simulink model "MMC_Per_arm_outer_v5_G2_case1b_delay02_aligned"  (R2024a)
settings: Solver=FixedStepDiscrete  StartTime=0.0  StopTime=2  FixedStep=Ts  RelTol=1e-3
PreLoadFcn:
  | % ---- MMC_Inner4 workspace parameters (control gains live inside the MATLAB Function blocks) ----
  | % ---------------- Converter ----------------
  | VDC     = 800;                  % DC-link voltage (V)  -> Vdc_pos / Vdc_neg = VDC/2
  | N       = 8;                    % submodules per arm
  | C       = 2.2e-3;               % submodule capacitance (F)  -> HB_xx blocks
  | vo      = 100;                  % nominal = initial capacitor voltage (V) = VDC/N  -> HB_xx, Vc_nom
  | W_nom   = 0.5*C*N*vo^2;         % nominal arm energy (J) -> initial condition of the Comm delay blocks
  | Larm    = 5e-3;                 % arm inductance (H)
  | Rarm    = 0.5;                  % arm resistance (ohm)
  | 
  | % ---------------- Grid and PCC filter ----------------
  | f       = 50;                   % grid frequency (Hz)
  | Vg_rms  = 230;                  % grid RMS voltage (V)
  | Vg_pk   = Vg_rms*sqrt(2);       % grid peak voltage (V) -> AC Voltage Source
  | Lg      = 2e-3;                 % line inductance (H)
  | Rg      = 0.1;                  % line resistance (ohm)
  | Cf      = 10e-6;                % AC filter capacitance (F)
  | Rf      = 10;                   % AC filter damping resistance (ohm)
  | 
  | % ---------------- Power set-points ----------------
  | Pstar   = 1500;                 % active-power set-point (W)
  | Qstar   = 0;                    % reactive-power set-point (var)
  | 
  | % ---------------- Timing ----------------
  | fsw     = 1250;                 % carrier frequency per submodule (Hz) -> N*fsw = 10 kHz per arm
  | Ts      = 1e-5;                 % simulation step = submodule-layer step (s)
  | Ts_ctrl = 1e-4;                 % arm-leader control step (s)
  | % ---------------- Test schedule: P* staircase and PCC load (added in _tests) ----------------
  | P_base   = 1500;                % staircase base = first level (W)
  | dP_step  = 250;                 % staircase step (W): 1500 -> 1750 -> 2000 -> 2250 -> 2500
  | t_step   = [0.6 1.0 1.4 1.8];   % step instants (s), 0.4 s hold at each level
  | t_back   = 2.2;                 % return to P_base (s) before the load test
  | P_load1  = 1000;                % PCC load 1 (W at 230 V rms)
  | P_load2  = 1000;                % PCC load 2 (W at 230 V rms)
  | R_load1  = Vg_rms^2/P_load1;    % 52.9 ohm
  | R_load2  = Vg_rms^2/P_load2;    % 52.9 ohm
  | t_load1  = 2.4;                 % Breaker load 1: closes at 2.4 s (stays closed)
  | t_load2  = [2.7 3.0];           % Breaker load 2: closes at 2.7 s, opens at 3.0 s
  | % ---- CASE: twin of case 1 with k_v = 0.2 (balanced start, P* fixed 1500 W, no PCC load, 2 s)
  | % ---- DERIVED: case1b_delay02_aligned: twin + own sample AND neighbour links delayed by 20 samples (0.2 ms), time-aligned
  | % P_SLEW = 5000 W/s, I_max = 17 A, P_max = 2500 W are set INSIDE mmc_outer_ctrl (both arm leaders)
  | t_load1  = 10;  t_load2 = [10 11];   % PCC load test disabled in this case (beyond StopTime)
InitFcn:
  | % ---- MMC_Inner4 workspace parameters (control gains live inside the MATLAB Function blocks) ----
  | % ---------------- Converter ----------------
  | VDC     = 800;                  % DC-link voltage (V)  -> Vdc_pos / Vdc_neg = VDC/2
  | N       = 8;                    % submodules per arm
  | C       = 2.2e-3;               % submodule capacitance (F)  -> HB_xx blocks
  | vo      = 100;                  % nominal = initial capacitor voltage (V) = VDC/N  -> HB_xx, Vc_nom
  | W_nom   = 0.5*C*N*vo^2;         % nominal arm energy (J) -> initial condition of the Comm delay blocks
  | Larm    = 5e-3;                 % arm inductance (H)
  | Rarm    = 0.5;                  % arm resistance (ohm)
  | 
  | % ---------------- Grid and PCC filter ----------------
  | f       = 50;                   % grid frequency (Hz)
  | Vg_rms  = 230;                  % grid RMS voltage (V)
  | Vg_pk   = Vg_rms*sqrt(2);       % grid peak voltage (V) -> AC Voltage Source
  | Lg      = 2e-3;                 % line inductance (H)
  | Rg      = 0.1;                  % line resistance (ohm)
  | Cf      = 10e-6;                % AC filter capacitance (F)
  | Rf      = 10;                   % AC filter damping resistance (ohm)
  | 
  | % ---------------- Power set-points ----------------
  | Pstar   = 1500;                 % active-power set-point (W)
  | Qstar   = 0;                    % reactive-power set-point (var)
  | 
  | % ---------------- Timing ----------------
  | fsw     = 1250;                 % carrier frequency per submodule (Hz) -> N*fsw = 10 kHz per arm
  | Ts      = 1e-5;                 % simulation step = submodule-layer step (s)
  | Ts_ctrl = 1e-4;                 % arm-leader control step (s)
  | % ---------------- Test schedule: P* staircase and PCC load (added in _tests) ----------------
  | P_base   = 1500;                % staircase base = first level (W)
  | dP_step  = 250;                 % staircase step (W): 1500 -> 1750 -> 2000 -> 2250 -> 2500
  | t_step   = [0.6 1.0 1.4 1.8];   % step instants (s), 0.4 s hold at each level
  | t_back   = 2.2;                 % return to P_base (s) before the load test
  | P_load1  = 1000;                % PCC load 1 (W at 230 V rms)
  | P_load2  = 1000;                % PCC load 2 (W at 230 V rms)
  | R_load1  = Vg_rms^2/P_load1;    % 52.9 ohm
  | R_load2  = Vg_rms^2/P_load2;    % 52.9 ohm
  | t_load1  = 2.4;                 % Breaker load 1: closes at 2.4 s (stays closed)
  | t_load2  = [2.7 3.0];           % Breaker load 2: closes at 2.7 s, opens at 3.0 s
  | % ---- CASE: twin of case 1 with k_v = 0.2 (balanced start, P* fixed 1500 W, no PCC load, 2 s)
  | % ---- DERIVED: case1b_delay02_aligned: twin + own sample AND neighbour links delayed by 20 samples (0.2 ms), time-aligned
  | % P_SLEW = 5000 W/s, I_max = 17 A, P_max = 2500 W are set INSIDE mmc_outer_ctrl (both arm leaders)
  | t_load1  = 10;  t_load2 = [10 11];   % PCC load test disabled in this case (beyond StopTime)
libraries: spsHalfBridgeMMCLib x16, spsSeriesRLCBranchLib x6, spsCurrentMeasurementLib x5, spsBreakerLib x2, spsGroundLib x2, spsDCVoltageSourceLib x2, spsACVoltageSourceLib x1, spspowerguiLib x1, spsVoltageMeasurementLib x1
(part 2 of 6)

== matlab function MMC_Per_arm_outer_v5_G2_case1b_delay02_aligned/SM_l3/Neighbors ==
  data: Vc_arm input; Vc_i output; i input; Vc_prev output; Vc_next output
function [Vc_i, Vc_prev, Vc_next] = get_neighbors(Vc_arm, i)
%#codegen
% =========================================================================
% GET_NEIGHBORS  -  Ring-link emulation for submodule number i
% -------------------------------------------------------------------------
% Block     : "Neighbors" inside every SM_ux / SM_lx subsystem
% Rate      : Ts = 10 us
% Instances : 16 (one per submodule)
% Purpose   : in simulation the whole capacitor-voltage vector of the arm is
%             available, but a real submodule only knows its OWN voltage and
%             the voltages of its two ring neighbours. This block hides
%             everything else, so the local controller stays truly local.
% Inputs    : Vc_arm  N x 1 vector of capacitor voltages of the arm (V)
%             i       own submodule index, 1..N
% Outputs   : Vc_i    own capacitor voltage (V)
%             Vc_prev voltage of the previous ring neighbour (V)
%             Vc_next voltage of the next ring neighbour (V)
% =========================================================================

%% ---------------- PARAMETERS ----------------
N = 8;                                   % submodules per arm (= length of Vc_arm, the Mux of the 8 HB voltages)
ND = 20;                              % ALIGNED-DELAY case: own AND neighbour values delayed by ND samples (Ts = 10 us -> 0.2 ms)
persistent buf_i buf_p buf_n idx         % circular buffers of the own sample and the two neighbour links, and the index

%% ---------------- 1. own index, made safe ----------------
k = min(max(round(i), 1), N);            % round to an integer and clamp to [1, N] (protects against a bad sm_id)

%% ---------------- 2. own voltage ----------------
Vc_i = Vc_arm(k);                        % own capacitor voltage

%% ---------------- 3. ring neighbours (circular: SM1 and SMN are neighbours) ----------------
if k == 1                                % first submodule of the ring
    Vc_prev = Vc_arm(N);                 % previous neighbour wraps around to the last submodule
    Vc_next = Vc_arm(2);                 % next neighbour is SM2
elseif k == N                            % last submodule of the ring
    Vc_prev = Vc_arm(N - 1);             % previous neighbour is SM(N-1)
    Vc_next = Vc_arm(1);                 % next neighbour wraps around to SM1
else                                     % any submodule in the middle
    Vc_prev = Vc_arm(k - 1);             % previous neighbour
    Vc_next = Vc_arm(k + 1);             % next neighbour
end

%% ---------------- 4. time-aligned delay: own sample and neighbour links delayed by the same ND (ALIGNED-DELAY case) ----------------
if isempty(buf_i)                        % first call
    buf_i = Vc_i    * ones(ND, 1);       % buffers start filled with the first values: no false error during the first ND samples
    buf_p = Vc_prev * ones(ND, 1);
    buf_n = Vc_next * ones(ND, 1);
    idx   = 1;
end
d_i    = buf_i(idx);                     % own voltage ND samples ago (same instant as the neighbour values)
d_prev = buf_p(idx);                     % value sent by the previous neighbour ND samples ago
d_next = buf_n(idx);                     % value sent by the next neighbour ND samples ago
buf_i(idx) = Vc_i;                       % store the fresh values in the slot just read
buf_p(idx) = Vc_prev;
buf_n(idx) = Vc_next;
idx = idx + 1;                           % advance the circular index
if idx > ND
    idx = 1;
end
Vc_i    = d_i;                           % the local controller compares three values of the SAME instant t - tau
Vc_prev = d_prev;
Vc_next = d_next;
end

== matlab function MMC_Per_arm_outer_v5_G2_case1b_delay02_aligned/SM_l3/Local Ctrl ==
  data: sm_id input; S_top output; m_arm input; i_arm input; Vc_i input; Vc_prev input; Vc_next input; t input; S_bot output
function [S_top, S_bot] = hb_sm_local_ctrl(sm_id, m_arm, i_arm, Vc_i, Vc_prev, Vc_next, t)
%#codegen
% =========================================================================
% HB_SM_LOCAL_CTRL  -  Submodule local controller: neighbour balancing + PSC-PWM
% -------------------------------------------------------------------------
% Block     : "Local Ctrl" inside every SM_ux / SM_lx subsystem
% Rate      : Ts = 10 us
% Instances : 16 (one per half-bridge submodule)
% Purpose   : decide the two gate signals of ONE half-bridge submodule using
%             only local information: own capacitor voltage, the two ring
%             neighbours, the arm modulation index sent by the arm leader,
%             the arm-current direction and the time base.
%             No sorting and no access to the full capacitor-voltage vector.
% Inputs    : sm_id    own index 1..N (sets the carrier phase shift)
%             m_arm    arm modulation index from the arm leader, in [0, 1]
%             i_arm    arm current (A), only its direction is used
%             Vc_i     own capacitor voltage (V)
%             Vc_prev  previous ring neighbour voltage (V)
%             Vc_next  next ring neighbour voltage (V)
%             t        simulation time (s), carrier time base
% Outputs   : S_top    upper switch gate (1 = on)  -> capacitor INSERTED (+Vc)
%             S_bot    lower switch gate (1 = on)  -> capacitor BYPASSED (0 V)
% =========================================================================

%% ---------------- PARAMETERS ----------------
N      = 8;                              % submodules per arm -> carrier phase shift of SM k = (k-1)/N of a period
fsw    = 1250;                           % carrier frequency per submodule (Hz) -> N*fsw = 10 kHz apparent arm ripple
k_v    = 0.2;                            % balancing gain (1/V): modulation-index change per volt of error
dead   = 0.1;                            % dead-band (V): errors smaller than this are ignored (no chattering)
Iscale = 1.0;                            % current scale (A) of the smooth sign function tanh(i_arm/Iscale)

%% ---------------- 1. neighbour-average balancing correction ----------------
err  = 0.5*(Vc_prev + Vc_next) - Vc_i;   % error = neighbour average - own voltage (> 0: I am too low, I need charging)
if abs(err) < dead                       % error inside the dead-band?
    err = 0;                             % ignore it
end
dirn = tanh(i_arm / Iscale);             % smooth current direction in (-1, +1); > 0 means inserting CHARGES the capacitor
dm   = k_v * err * dirn;                 % correction: insert more if charging is needed AND the current charges, less otherwise
m_i  = min(max(m_arm + dm, 0), 1);       % own modulation index = arm index + correction, clamped to [0, 1]

%% ---------------- 2. phase-shifted triangular carrier (0 -> 1 -> 0) ----------------
tau = mod(t*fsw + (sm_id - 1)/N, 1);     % position inside the carrier period, in [0, 1), shifted by (sm_id-1)/N
car = 1 - abs(2*tau - 1);                % triangle: rises 0 -> 1 on the first half, falls 1 -> 0 on the second half

%% ---------------- 3. half-bridge gating ----------------
if m_i >= car                            % modulation index above the carrier?
    S_top = 1;                           % upper switch on  -> capacitor inserted (+Vc on the arm)
    S_bot = 0;                           % lower switch off
else                                     % modulation index below the carrier
    S_top = 0;                           % upper switch off
    S_bot = 1;                           % lower switch on  -> capacitor bypassed (0 V)
end
end

== matlab function MMC_Per_arm_outer_v5_G2_case1b_delay02_aligned/SM_u4/Neighbors ==
  data: Vc_arm input; Vc_i output; i input; Vc_prev output; Vc_next output
function [Vc_i, Vc_prev, Vc_next] = get_neighbors(Vc_arm, i)
%#codegen
% =========================================================================
% GET_NEIGHBORS  -  Ring-link emulation for submodule number i
% -------------------------------------------------------------------------
% Block     : "Neighbors" inside every SM_ux / SM_lx subsystem
% Rate      : Ts = 10 us
% Instances : 16 (one per submodule)
% Purpose   : in simulation the whole capacitor-voltage vector of the arm is
%             available, but a real submodule only knows its OWN voltage and
%             the voltages of its two ring neighbours. This block hides
%             everything else, so the local controller stays truly local.
% Inputs    : Vc_arm  N x 1 vector of capacitor voltages of the arm (V)
%             i       own submodule index, 1..N
% Outputs   : Vc_i    own capacitor voltage (V)
%             Vc_prev voltage of the previous ring neighbour (V)
%             Vc_next voltage of the next ring neighbour (V)
% =========================================================================

%% ---------------- PARAMETERS ----------------
N = 8;                                   % submodules per arm (= length of Vc_arm, the Mux of the 8 HB voltages)
ND = 20;                              % ALIGNED-DELAY case: own AND neighbour values delayed by ND samples (Ts = 10 us -> 0.2 ms)
persistent buf_i buf_p buf_n idx         % circular buffers of the own sample and the two neighbour links, and the index

%% ---------------- 1. own index, made safe ----------------
k = min(max(round(i), 1), N);            % round to an integer and clamp to [1, N] (protects against a bad sm_id)

%% ---------------- 2. own voltage ----------------
Vc_i = Vc_arm(k);                        % own capacitor voltage

%% ---------------- 3. ring neighbours (circular: SM1 and SMN are neighbours) ----------------
if k == 1                                % first submodule of the ring
    Vc_prev = Vc_arm(N);                 % previous neighbour wraps around to the last submodule
    Vc_next = Vc_arm(2);                 % next neighbour is SM2
elseif k == N                            % last submodule of the ring
    Vc_prev = Vc_arm(N - 1);             % previous neighbour is SM(N-1)
    Vc_next = Vc_arm(1);                 % next neighbour wraps around to SM1
else                                     % any submodule in the middle
    Vc_prev = Vc_arm(k - 1);             % previous neighbour
    Vc_next = Vc_arm(k + 1);             % next neighbour
end

%% ---------------- 4. time-aligned delay: own sample and neighbour links delayed by the same ND (ALIGNED-DELAY case) ----------------
if isempty(buf_i)                        % first call
    buf_i = Vc_i    * ones(ND, 1);       % buffers start filled with the first values: no false error during the first ND samples
    buf_p = Vc_prev * ones(ND, 1);
    buf_n = Vc_next * ones(ND, 1);
    idx   = 1;
end
d_i    = buf_i(idx);                     % own voltage ND samples ago (same instant as the neighbour values)
d_prev = buf_p(idx);                     % value sent by the previous neighbour ND samples ago
d_next = buf_n(idx);                     % value sent by the next neighbour ND samples ago
buf_i(idx) = Vc_i;                       % store the fresh values in the slot just read
buf_p(idx) = Vc_prev;
buf_n(idx) = Vc_next;
idx = idx + 1;                           % advance the circular index
if idx > ND
    idx = 1;
end
Vc_i    = d_i;                           % the local controller compares three values of the SAME instant t - tau
Vc_prev = d_prev;
Vc_next = d_next;
end

== matlab function MMC_Per_arm_outer_v5_G2_case1b_delay02_aligned/SM_u1/Local Ctrl ==
  data: sm_id input; S_top output; m_arm input; i_arm input; Vc_i input; Vc_prev input; Vc_next input; t input; S_bot output
function [S_top, S_bot] = hb_sm_local_ctrl(sm_id, m_arm, i_arm, Vc_i, Vc_prev, Vc_next, t)
%#codegen
% =========================================================================
% HB_SM_LOCAL_CTRL  -  Submodule local controller: neighbour balancing + PSC-PWM
% -------------------------------------------------------------------------
% Block     : "Local Ctrl" inside every SM_ux / SM_lx subsystem
% Rate      : Ts = 10 us
% Instances : 16 (one per half-bridge submodule)
% Purpose   : decide the two gate signals of ONE half-bridge submodule using
%             only local information: own capacitor voltage, the two ring
%             neighbours, the arm modulation index sent by the arm leader,
%             the arm-current direction and the time base.
%             No sorting and no access to the full capacitor-voltage vector.
% Inputs    : sm_id    own index 1..N (sets the carrier phase shift)
%             m_arm    arm modulation index from the arm leader, in [0, 1]
%             i_arm    arm current (A), only its direction is used
%             Vc_i     own capacitor voltage (V)
%             Vc_prev  previous ring neighbour voltage (V)
%             Vc_next  next ring neighbour voltage (V)
%             t        simulation time (s), carrier time base
% Outputs   : S_top    upper switch gate (1 = on)  -> capacitor INSERTED (+Vc)
%             S_bot    lower switch gate (1 = on)  -> capacitor BYPASSED (0 V)
% =========================================================================

%% ---------------- PARAMETERS ----------------
N      = 8;                              % submodules per arm -> carrier phase shift of SM k = (k-1)/N of a period
fsw    = 1250;                           % carrier frequency per submodule (Hz) -> N*fsw = 10 kHz apparent arm ripple
k_v    = 0.2;                            % balancing gain (1/V): modulation-index change per volt of error
dead   = 0.1;                            % dead-band (V): errors smaller than this are ignored (no chattering)
Iscale = 1.0;                            % current scale (A) of the smooth sign function tanh(i_arm/Iscale)

%% ---------------- 1. neighbour-average balancing correction ----------------
err  = 0.5*(Vc_prev + Vc_next) - Vc_i;   % error = neighbour average - own voltage (> 0: I am too low, I need charging)
if abs(err) < dead                       % error inside the dead-band?
    err = 0;                             % ignore it
end
dirn = tanh(i_arm / Iscale);             % smooth current direction in (-1, +1); > 0 means inserting CHARGES the capacitor
dm   = k_v * err * dirn;                 % correction: insert more if charging is needed AND the current charges, less otherwise
m_i  = min(max(m_arm + dm, 0), 1);       % own modulation index = arm index + correction, clamped to [0, 1]

%% ---------------- 2. phase-shifted triangular carrier (0 -> 1 -> 0) ----------------
tau = mod(t*fsw + (sm_id - 1)/N, 1);     % position inside the carrier period, in [0, 1), shifted by (sm_id-1)/N
car = 1 - abs(2*tau - 1);                % triangle: rises 0 -> 1 on the first half, falls 1 -> 0 on the second half

%% ---------------- 3. half-bridge gating ----------------
if m_i >= car                            % modulation index above the carrier?
    S_top = 1;                           % upper switch on  -> capacitor inserted (+Vc on the arm)
    S_bot = 0;                           % lower switch off
else                                     % modulation index below the carrier
    S_top = 0;                           % upper switch off
    S_bot = 1;                           % lower switch on  -> capacitor bypassed (0 V)
end
end

== matlab function MMC_Per_arm_outer_v5_G2_case1b_delay02_aligned/SM_u4/Local Ctrl ==
  data: sm_id input; S_top output; m_arm input; i_arm input; Vc_i input; Vc_prev input; Vc_next input; t input; S_bot output
function [S_top, S_bot] = hb_sm_local_ctrl(sm_id, m_arm, i_arm, Vc_i, Vc_prev, Vc_next, t)
%#codegen
% =========================================================================
% HB_SM_LOCAL_CTRL  -  Submodule local controller: neighbour balancing + PSC-PWM
% -------------------------------------------------------------------------
% Block     : "Local Ctrl" inside every SM_ux / SM_lx subsystem
% Rate      : Ts = 10 us
% Instances : 16 (one per half-bridge submodule)
% Purpose   : decide the two gate signals of ONE half-bridge submodule using
%             only local information: own capacitor voltage, the two ring
%             neighbours, the arm modulation index sent by the arm leader,
%             the arm-current direction and the time base.
%             No sorting and no access to the full capacitor-voltage vector.
% Inputs    : sm_id    own index 1..N (sets the carrier phase shift)
%             m_arm    arm modulation index from the arm leader, in [0, 1]
%             i_arm    arm current (A), only its direction is used
%             Vc_i     own capacitor voltage (V)
%             Vc_prev  previous ring neighbour voltage (V)
%             Vc_next  next ring neighbour voltage (V)
%             t        simulation time (s), carrier time base
% Outputs   : S_top    upper switch gate (1 = on)  -> capacitor INSERTED (+Vc)
%             S_bot    lower switch gate (1 = on)  -> capacitor BYPASSED (0 V)
% =========================================================================

%% ---------------- PARAMETERS ----------------
N      = 8;                              % submodules per arm -> carrier phase shift of SM k = (k-1)/N of a period
fsw    = 1250;                           % carrier frequency per submodule (Hz) -> N*fsw = 10 kHz apparent arm ripple
k_v    = 0.2;                            % balancing gain (1/V): modulation-index change per volt of error
dead   = 0.1;                            % dead-band (V): errors smaller than this are ignored (no chattering)
Iscale = 1.0;                            % current scale (A) of the smooth sign function tanh(i_arm/Iscale)

%% ---------------- 1. neighbour-average balancing correction ----------------
err  = 0.5*(Vc_prev + Vc_next) - Vc_i;   % error = neighbour average - own voltage (> 0: I am too low, I need charging)
if abs(err) < dead                       % error inside the dead-band?
    err = 0;                             % ignore it
end
dirn = tanh(i_arm / Iscale);             % smooth current direction in (-1, +1); > 0 means inserting CHARGES the capacitor
dm   = k_v * err * dirn;                 % correction: insert more if charging is needed AND the current charges, less otherwise
m_i  = min(max(m_arm + dm, 0), 1);       % own modulation index = arm index + correction, clamped to [0, 1]

%% ---------------- 2. phase-shifted triangular carrier (0 -> 1 -> 0) ----------------
tau = mod(t*fsw + (sm_id - 1)/N, 1);     % position inside the carrier period, in [0, 1), shifted by (sm_id-1)/N
car = 1 - abs(2*tau - 1);                % triangle: rises 0 -> 1 on the first half, falls 1 -> 0 on the second half

%% ---------------- 3. half-bridge gating ----------------
if m_i >= car                            % modulation index above the carrier?
    S_top = 1;                           % upper switch on  -> capacitor inserted (+Vc on the arm)
    S_bot = 0;                           % lower switch off
else                                     % modulation index below the carrier
    S_top = 0;                           % upper switch off
    S_bot = 1;                           % lower switch on  -> capacitor bypassed (0 V)
end
end

== matlab function MMC_Per_arm_outer_v5_G2_case1b_delay02_aligned/SM_l4/Neighbors ==
  data: Vc_arm input; Vc_i output; i input; Vc_prev output; Vc_next output
function [Vc_i, Vc_prev, Vc_next] = get_neighbors(Vc_arm, i)
%#codegen
% =========================================================================
% GET_NEIGHBORS  -  Ring-link emulation for submodule number i
% -------------------------------------------------------------------------
% Block     : "Neighbors" inside every SM_ux / SM_lx subsystem
% Rate      : Ts = 10 us
% Instances : 16 (one per submodule)
% Purpose   : in simulation the whole capacitor-voltage vector of the arm is
%             available, but a real submodule only knows its OWN voltage and
%             the voltages of its two ring neighbours. This block hides
%             everything else, so the local controller stays truly local.
% Inputs    : Vc_arm  N x 1 vector of capacitor voltages of the arm (V)
%             i       own submodule index, 1..N
% Outputs   : Vc_i    own capacitor voltage (V)
%             Vc_prev voltage of the previous ring neighbour (V)
%             Vc_next voltage of the next ring neighbour (V)
% =========================================================================

%% ---------------- PARAMETERS ----------------
N = 8;                                   % submodules per arm (= length of Vc_arm, the Mux of the 8 HB voltages)
ND = 20;                              % ALIGNED-DELAY case: own AND neighbour values delayed by ND samples (Ts = 10 us -> 0.2 ms)
persistent buf_i buf_p buf_n idx         % circular buffers of the own sample and the two neighbour links, and the index

%% ---------------- 1. own index, made safe ----------------
k = min(max(round(i), 1), N);            % round to an integer and clamp to [1, N] (protects against a bad sm_id)

%% ---------------- 2. own voltage ----------------
Vc_i = Vc_arm(k);                        % own capacitor voltage

%% ---------------- 3. ring neighbours (circular: SM1 and SMN are neighbours) ----------------
if k == 1                                % first submodule of the ring
    Vc_prev = Vc_arm(N);                 % previous neighbour wraps around to the last submodule
    Vc_next = Vc_arm(2);                 % next neighbour is SM2
elseif k == N                            % last submodule of the ring
    Vc_prev = Vc_arm(N - 1);             % previous neighbour is SM(N-1)
    Vc_next = Vc_arm(1);                 % next neighbour wraps around to SM1
else                                     % any submodule in the middle
    Vc_prev = Vc_arm(k - 1);             % previous neighbour
    Vc_next = Vc_arm(k + 1);             % next neighbour
end

%% ---------------- 4. time-aligned delay: own sample and neighbour links delayed by the same ND (ALIGNED-DELAY case) ----------------
if isempty(buf_i)                        % first call
    buf_i = Vc_i    * ones(ND, 1);       % buffers start filled with the first values: no false error during the first ND samples
    buf_p = Vc_prev * ones(ND, 1);
    buf_n = Vc_next * ones(ND, 1);
    idx   = 1;
end
d_i    = buf_i(idx);                     % own voltage ND samples ago (same instant as the neighbour values)
d_prev = buf_p(idx);                     % value sent by the previous neighbour ND samples ago
d_next = buf_n(idx);                     % value sent by the next neighbour ND samples ago
buf_i(idx) = Vc_i;                       % store the fresh values in the slot just read
buf_p(idx) = Vc_prev;
buf_n(idx) = Vc_next;
idx = idx + 1;                           % advance the circular index
if idx > ND
    idx = 1;
end
Vc_i    = d_i;                           % the local controller compares three values of the SAME instant t - tau
Vc_prev = d_prev;
Vc_next = d_next;
end

== matlab function MMC_Per_arm_outer_v5_G2_case1b_delay02_aligned/SM_l4/Local Ctrl ==
  data: sm_id input; S_top output; m_arm input; i_arm input; Vc_i input; Vc_prev input; Vc_next input; t input; S_bot output
function [S_top, S_bot] = hb_sm_local_ctrl(sm_id, m_arm, i_arm, Vc_i, Vc_prev, Vc_next, t)
%#codegen
% =========================================================================
% HB_SM_LOCAL_CTRL  -  Submodule local controller: neighbour balancing + PSC-PWM
% -------------------------------------------------------------------------
% Block     : "Local Ctrl" inside every SM_ux / SM_lx subsystem
% Rate      : Ts = 10 us
% Instances : 16 (one per half-bridge submodule)
% Purpose   : decide the two gate signals of ONE half-bridge submodule using
%             only local information: own capacitor voltage, the two ring
%             neighbours, the arm modulation index sent by the arm leader,
%             the arm-current direction and the time base.
%             No sorting and no access to the full capacitor-voltage vector.
% Inputs    : sm_id    own index 1..N (sets the carrier phase shift)
%             m_arm    arm modulation index from the arm leader, in [0, 1]
%             i_arm    arm current (A), only its direction is used
%             Vc_i     own capacitor voltage (V)
%             Vc_prev  previous ring neighbour voltage (V)
%             Vc_next  next ring neighbour voltage (V)
%             t        simulation time (s), carrier time base
% Outputs   : S_top    upper switch gate (1 = on)  -> capacitor INSERTED (+Vc)
%             S_bot    lower switch gate (1 = on)  -> capacitor BYPASSED (0 V)
% =========================================================================

%% ---------------- PARAMETERS ----------------
N      = 8;                              % submodules per arm -> carrier phase shift of SM k = (k-1)/N of a period
fsw    = 1250;                           % carrier frequency per submodule (Hz) -> N*fsw = 10 kHz apparent arm ripple
k_v    = 0.2;                            % balancing gain (1/V): modulation-index change per volt of error
dead   = 0.1;                            % dead-band (V): errors smaller than this are ignored (no chattering)
Iscale = 1.0;                            % current scale (A) of the smooth sign function tanh(i_arm/Iscale)

%% ---------------- 1. neighbour-average balancing correction ----------------
err  = 0.5*(Vc_prev + Vc_next) - Vc_i;   % error = neighbour average - own voltage (> 0: I am too low, I need charging)
if abs(err) < dead                       % error inside the dead-band?
    err = 0;                             % ignore it
end
dirn = tanh(i_arm / Iscale);             % smooth current direction in (-1, +1); > 0 means inserting CHARGES the capacitor
dm   = k_v * err * dirn;                 % correction: insert more if charging is needed AND the current charges, less otherwise
m_i  = min(max(m_arm + dm, 0), 1);       % own modulation index = arm index + correction, clamped to [0, 1]

%% ---------------- 2. phase-shifted triangular carrier (0 -> 1 -> 0) ----------------
tau = mod(t*fsw + (sm_id - 1)/N, 1);     % position inside the carrier period, in [0, 1), shifted by (sm_id-1)/N
car = 1 - abs(2*tau - 1);                % triangle: rises 0 -> 1 on the first half, falls 1 -> 0 on the second half

%% ---------------- 3. half-bridge gating ----------------
if m_i >= car                            % modulation index above the carrier?
    S_top = 1;                           % upper switch on  -> capacitor inserted (+Vc on the arm)
    S_bot = 0;                           % lower switch off
else                                     % modulation index below the carrier
    S_top = 0;                           % upper switch off
    S_bot = 1;                           % lower switch on  -> capacitor bypassed (0 V)
end
end

== matlab function MMC_Per_arm_outer_v5_G2_case1b_delay02_aligned/SM_u5/Neighbors ==
  data: Vc_arm input; Vc_i output; i input; Vc_prev output; Vc_next output
function [Vc_i, Vc_prev, Vc_next] = get_neighbors(Vc_arm, i)
%#codegen
% =========================================================================
% GET_NEIGHBORS  -  Ring-link emulation for submodule number i
% -------------------------------------------------------------------------
% Block     : "Neighbors" inside every SM_ux / SM_lx subsystem
% Rate      : Ts = 10 us
% Instances : 16 (one per submodule)
% Purpose   : in simulation the whole capacitor-voltage vector of the arm is
%             available, but a real submodule only knows its OWN voltage and
%             the voltages of its two ring neighbours. This block hides
%             everything else, so the local controller stays truly local.
% Inputs    : Vc_arm  N x 1 vector of capacitor voltages of the arm (V)
%             i       own submodule index, 1..N
% Outputs   : Vc_i    own capacitor voltage (V)
%             Vc_prev voltage of the previous ring neighbour (V)
%             Vc_next voltage of the next ring neighbour (V)
% =========================================================================

%% ---------------- PARAMETERS ----------------
N = 8;                                   % submodules per arm (= length of Vc_arm, the Mux of the 8 HB voltages)
ND = 20;                              % ALIGNED-DELAY case: own AND neighbour values delayed by ND samples (Ts = 10 us -> 0.2 ms)
persistent buf_i buf_p buf_n idx         % circular buffers of the own sample and the two neighbour links, and the index

%% ---------------- 1. own index, made safe ----------------
k = min(max(round(i), 1), N);            % round to an integer and clamp to [1, N] (protects against a bad sm_id)

%% ---------------- 2. own voltage ----------------
Vc_i = Vc_arm(k);                        % own capacitor voltage

%% ---------------- 3. ring neighbours (circular: SM1 and SMN are neighbours) ----------------
if k == 1                                % first submodule of the ring
    Vc_prev = Vc_arm(N);                 % previous neighbour wraps around to the last submodule
    Vc_next = Vc_arm(2);                 % next neighbour is SM2
elseif k == N                            % last submodule of the ring
    Vc_prev = Vc_arm(N - 1);             % previous neighbour is SM(N-1)
    Vc_next = Vc_arm(1);                 % next neighbour wraps around to SM1
else                                     % any submodule in the middle
    Vc_prev = Vc_arm(k - 1);             % previous neighbour
    Vc_next = Vc_arm(k + 1);             % next neighbour
end

%% ---------------- 4. time-aligned delay: own sample and neighbour links delayed by the same ND (ALIGNED-DELAY case) ----------------
if isempty(buf_i)                        % first call
    buf_i = Vc_i    * ones(ND, 1);       % buffers start filled with the first values: no false error during the first ND samples
    buf_p = Vc_prev * ones(ND, 1);
    buf_n = Vc_next * ones(ND, 1);
    idx   = 1;
end
d_i    = buf_i(idx);                     % own voltage ND samples ago (same instant as the neighbour values)
d_prev = buf_p(idx);                     % value sent by the previous neighbour ND samples ago
d_next = buf_n(idx);                     % value sent by the next neighbour ND samples ago
buf_i(idx) = Vc_i;                       % store the fresh values in the slot just read
buf_p(idx) = Vc_prev;
buf_n(idx) = Vc_next;
idx = idx + 1;                           % advance the circular index
if idx > ND
    idx = 1;
end
Vc_i    = d_i;                           % the local controller compares three values of the SAME instant t - tau
Vc_prev = d_prev;
Vc_next = d_next;
end

== matlab function MMC_Per_arm_outer_v5_G2_case1b_delay02_aligned/SM_u5/Local Ctrl ==
  data: sm_id input; S_top output; m_arm input; i_arm input; Vc_i input; Vc_prev input; Vc_next input; t input; S_bot output
function [S_top, S_bot] = hb_sm_local_ctrl(sm_id, m_arm, i_arm, Vc_i, Vc_prev, Vc_next, t)
%#codegen
% =========================================================================
% HB_SM_LOCAL_CTRL  -  Submodule local controller: neighbour balancing + PSC-PWM
% -------------------------------------------------------------------------
% Block     : "Local Ctrl" inside every SM_ux / SM_lx subsystem
% Rate      : Ts = 10 us
% Instances : 16 (one per half-bridge submodule)
% Purpose   : decide the two gate signals of ONE half-bridge submodule using
%             only local information: own capacitor voltage, the two ring
%             neighbours, the arm modulation index sent by the arm leader,
%             the arm-current direction and the time base.
%             No sorting and no access to the full capacitor-voltage vector.
% Inputs    : sm_id    own index 1..N (sets the carrier phase shift)
%             m_arm    arm modulation index from the arm leader, in [0, 1]
%             i_arm    arm current (A), only its direction is used
%             Vc_i     own capacitor voltage (V)
%             Vc_prev  previous ring neighbour voltage (V)
%             Vc_next  next ring neighbour voltage (V)
%             t        simulation time (s), carrier time base
% Outputs   : S_top    upper switch gate (1 = on)  -> capacitor INSERTED (+Vc)
%             S_bot    lower switch gate (1 = on)  -> capacitor BYPASSED (0 V)
% =========================================================================

%% ---------------- PARAMETERS ----------------
N      = 8;                              % submodules per arm -> carrier phase shift of SM k = (k-1)/N of a period
fsw    = 1250;                           % carrier frequency per submodule (Hz) -> N*fsw = 10 kHz apparent arm ripple
k_v    = 0.2;                            % balancing gain (1/V): modulation-index change per volt of error
dead   = 0.1;                            % dead-band (V): errors smaller than this are ignored (no chattering)
Iscale = 1.0;                            % current scale (A) of the smooth sign function tanh(i_arm/Iscale)

%% ---------------- 1. neighbour-average balancing correction ----------------
err  = 0.5*(Vc_prev + Vc_next) - Vc_i;   % error = neighbour average - own voltage (> 0: I am too low, I need charging)
if abs(err) < dead                       % error inside the dead-band?
    err = 0;                             % ignore it
end
dirn = tanh(i_arm / Iscale);             % smooth current direction in (-1, +1); > 0 means inserting CHARGES the capacitor
dm   = k_v * err * dirn;                 % correction: insert more if charging is needed AND the current charges, less otherwise
m_i  = min(max(m_arm + dm, 0), 1);       % own modulation index = arm index + correction, clamped to [0, 1]

%% ---------------- 2. phase-shifted triangular carrier (0 -> 1 -> 0) ----------------
tau = mod(t*fsw + (sm_id - 1)/N, 1);     % position inside the carrier period, in [0, 1), shifted by (sm_id-1)/N
car = 1 - abs(2*tau - 1);                % triangle: rises 0 -> 1 on the first half, falls 1 -> 0 on the second half

%% ---------------- 3. half-bridge gating ----------------
if m_i >= car                            % modulation index above the carrier?
    S_top = 1;                           % upper switch on  -> capacitor inserted (+Vc on the arm)
    S_bot = 0;                           % lower switch off
else                                     % modulation index below the carrier
    S_top = 0;                           % upper switch off
    S_bot = 1;                           % lower switch on  -> capacitor bypassed (0 V)
end
end

== matlab function MMC_Per_arm_outer_v5_G2_case1b_delay02_aligned/SM_l5/Neighbors ==
  data: Vc_arm input; Vc_i output; i input; Vc_prev output; Vc_next output
function [Vc_i, Vc_prev, Vc_next] = get_neighbors(Vc_arm, i)
%#codegen
% =========================================================================
% GET_NEIGHBORS  -  Ring-link emulation for submodule number i
% -------------------------------------------------------------------------
% Block     : "Neighbors" inside every SM_ux / SM_lx subsystem
% Rate      : Ts = 10 us
% Instances : 16 (one per submodule)
% Purpose   : in simulation the whole capacitor-voltage vector of the arm is
%             available, but a real submodule only knows its OWN voltage and
%             the voltages of its two ring neighbours. This block hides
%             everything else, so the local controller stays truly local.
% Inputs    : Vc_arm  N x 1 vector of capacitor voltages of the arm (V)
%             i       own submodule index, 1..N
% Outputs   : Vc_i    own capacitor voltage (V)
%             Vc_prev voltage of the previous ring neighbour (V)
%             Vc_next voltage of the next ring neighbour (V)
% =========================================================================

%% ---------------- PARAMETERS ----------------
N = 8;                                   % submodules per arm (= length of Vc_arm, the Mux of the 8 HB voltages)
ND = 20;                              % ALIGNED-DELAY case: own AND neighbour values delayed by ND samples (Ts = 10 us -> 0.2 ms)
persistent buf_i buf_p buf_n idx         % circular buffers of the own sample and the two neighbour links, and the index

%% ---------------- 1. own index, made safe ----------------
k = min(max(round(i), 1), N);            % round to an integer and clamp to [1, N] (protects against a bad sm_id)

%% ---------------- 2. own voltage ----------------
Vc_i = Vc_arm(k);                        % own capacitor voltage

%% ---------------- 3. ring neighbours (circular: SM1 and SMN are neighbours) ----------------
if k == 1                                % first submodule of the ring
    Vc_prev = Vc_arm(N);                 % previous neighbour wraps around to the last submodule
    Vc_next = Vc_arm(2);                 % next neighbour is SM2
elseif k == N                            % last submodule of the ring
    Vc_prev = Vc_arm(N - 1);             % previous neighbour is SM(N-1)
    Vc_next = Vc_arm(1);                 % next neighbour wraps around to SM1
else                                     % any submodule in the middle
    Vc_prev = Vc_arm(k - 1);             % previous neighbour
    Vc_next = Vc_arm(k + 1);             % next neighbour
end

%% ---------------- 4. time-aligned delay: own sample and neighbour links delayed by the same ND (ALIGNED-DELAY case) ----------------
if isempty(buf_i)                        % first call
    buf_i = Vc_i    * ones(ND, 1);       % buffers start filled with the first values: no false error during the first ND samples
    buf_p = Vc_prev * ones(ND, 1);
    buf_n = Vc_next * ones(ND, 1);
    idx   = 1;
end
d_i    = buf_i(idx);                     % own voltage ND samples ago (same instant as the neighbour values)
d_prev = buf_p(idx);                     % value sent by the previous neighbour ND samples ago
d_next = buf_n(idx);                     % value sent by the next neighbour ND samples ago
buf_i(idx) = Vc_i;                       % store the fresh values in the slot just read
buf_p(idx) = Vc_prev;
buf_n(idx) = Vc_next;
idx = idx + 1;                           % advance the circular index
if idx > ND
    idx = 1;
end
Vc_i    = d_i;                           % the local controller compares three values of the SAME instant t - tau
Vc_prev = d_prev;
Vc_next = d_next;
end

== matlab function MMC_Per_arm_outer_v5_G2_case1b_delay02_aligned/SM_l5/Local Ctrl ==
  data: sm_id input; S_top output; m_arm input; i_arm input; Vc_i input; Vc_prev input; Vc_next input; t input; S_bot output
function [S_top, S_bot] = hb_sm_local_ctrl(sm_id, m_arm, i_arm, Vc_i, Vc_prev, Vc_next, t)
%#codegen
% =========================================================================
% HB_SM_LOCAL_CTRL  -  Submodule local controller: neighbour balancing + PSC-PWM
% -------------------------------------------------------------------------
% Block     : "Local Ctrl" inside every SM_ux / SM_lx subsystem
% Rate      : Ts = 10 us
% Instances : 16 (one per half-bridge submodule)
% Purpose   : decide the two gate signals of ONE half-bridge submodule using
%             only local information: own capacitor voltage, the two ring
%             neighbours, the arm modulation index sent by the arm leader,
%             the arm-current direction and the time base.
%             No sorting and no access to the full capacitor-voltage vector.
% Inputs    : sm_id    own index 1..N (sets the carrier phase shift)
%             m_arm    arm modulation index from the arm leader, in [0, 1]
%             i_arm    arm current (A), only its direction is used
%             Vc_i     own capacitor voltage (V)
%             Vc_prev  previous ring neighbour voltage (V)
%             Vc_next  next ring neighbour voltage (V)
%             t        simulation time (s), carrier time base
% Outputs   : S_top    upper switch gate (1 = on)  -> capacitor INSERTED (+Vc)
%             S_bot    lower switch gate (1 = on)  -> capacitor BYPASSED (0 V)
% =========================================================================

%% ---------------- PARAMETERS ----------------
N      = 8;                              % submodules per arm -> carrier phase shift of SM k = (k-1)/N of a period
fsw    = 1250;                           % carrier frequency per submodule (Hz) -> N*fsw = 10 kHz apparent arm ripple
k_v    = 0.2;                            % balancing gain (1/V): modulation-index change per volt of error
dead   = 0.1;                            % dead-band (V): errors smaller than this are ignored (no chattering)
Iscale = 1.0;                            % current scale (A) of the smooth sign function tanh(i_arm/Iscale)

%% ---------------- 1. neighbour-average balancing correction ----------------
err  = 0.5*(Vc_prev + Vc_next) - Vc_i;   % error = neighbour average - own voltage (> 0: I am too low, I need charging)
if abs(err) < dead                       % error inside the dead-band?
    err = 0;                             % ignore it
end
dirn = tanh(i_arm / Iscale);             % smooth current direction in (-1, +1); > 0 means inserting CHARGES the capacitor
dm   = k_v * err * dirn;                 % correction: insert more if charging is needed AND the current charges, less otherwise
m_i  = min(max(m_arm + dm, 0), 1);       % own modulation index = arm index + correction, clamped to [0, 1]

%% ---------------- 2. phase-shifted triangular carrier (0 -> 1 -> 0) ----------------
tau = mod(t*fsw + (sm_id - 1)/N, 1);     % position inside the carrier period, in [0, 1), shifted by (sm_id-1)/N
car = 1 - abs(2*tau - 1);                % triangle: rises 0 -> 1 on the first half, falls 1 -> 0 on the second half

%% ---------------- 3. half-bridge gating ----------------
if m_i >= car                            % modulation index above the carrier?
    S_top = 1;                           % upper switch on  -> capacitor inserted (+Vc on the arm)
    S_bot = 0;                           % lower switch off
else                                     % modulation index below the carrier
    S_top = 0;                           % upper switch off
    S_bot = 1;                           % lower switch on  -> capacitor bypassed (0 V)
end
end
